simulink model "TractorTransmissionTradeOff"  (R2025a)
settings: Solver=daessc  StartTime=0.0  StopTime=125  RelTol=1e-3  AbsTol=1e-3
PreLoadFcn:
  | distanceVector = [0,0.1389,0.4167,0.8333,1.3889,2.0833,2.9167,3.889,5,6.25,7.6389,200];
  | targetVelocityVector = [0,0.5,1,1.5,2,2.5,3,3.5,4,4.5,5,5];
InitFcn:
  | TractorEnergyComputationInput
undefined symbols (not defined in the file or in its folder): engine, implement, tc, tire, tk, tphi, tykc, tykphi, tyn
libraries: nesl_utility x33, fl_lib x18, sdl_lib x6, simulink x5, slpidlib x1
(part 3 of 3)

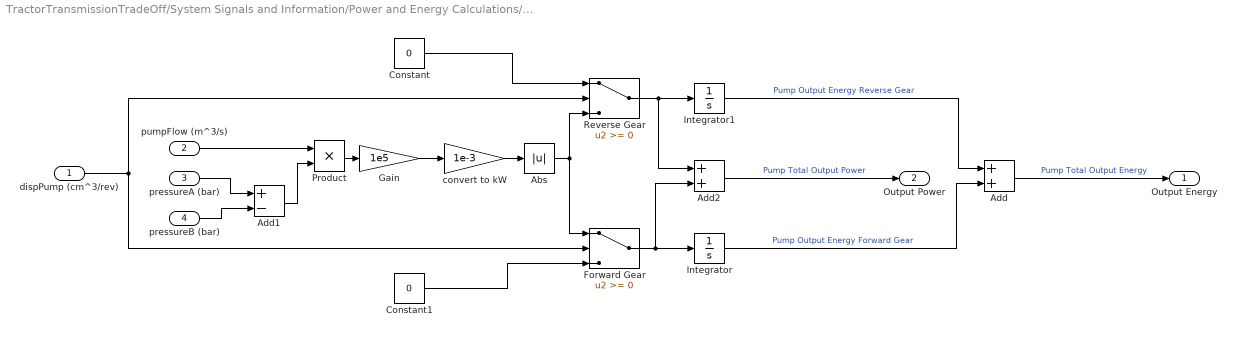
== system TractorTransmissionTradeOff/System Signals and Information/Power and Energy Calculations/Pump Computation/Pump Output Energy Computation ==
  dispPump (cm^3/rev) : Inport
  pumpFlow (m^3/s) : Inport  Port=2
  pressureA (bar) : Inport  Port=3
  pressureB (bar) : Inport  Port=4
  Abs : Abs  ZeroCross=off  SaturateOnIntegerOverflow=off
  Add : Sum
  Add1 : Sum  Inputs=+-
  Add2 : Sum
  Constant : Constant  Value=0
  Constant1 : Constant  Value=0
  Forward Gear : Switch  SaturateOnIntegerOverflow=off  InputSameDT=off
  Gain : Gain  Gain=1e5
  Integrator : Integrator
  Integrator1 : Integrator
  Product : Product
  Reverse Gear : Switch  SaturateOnIntegerOverflow=off  InputSameDT=off
  convert to kW : Gain  Gain=1e-3
  Output Energy : Outport
  Output Power : Outport  Port=2
  wires:
  pumpFlow (m^3/s)/1 -> Product/1
  Product/1 -> Gain/1
  dispPump (cm^3/rev)/1 -> Reverse Gear/2, Forward Gear/2
  Constant/1 -> Reverse Gear/1
  Constant1/1 -> Forward Gear/3
  Reverse Gear/1 -> Integrator1/1, Add2/1
  Forward Gear/1 -> Integrator/1, Add2/2
  Integrator1/1 -> Add/1  "Pump Output Energy Reverse Gear"
  Integrator/1 -> Add/2  "Pump Output Energy Forward Gear"
  Add/1 -> Output Energy/1  "Pump Total Output Energy"
  pressureA (bar)/1 -> Add1/1
  pressureB (bar)/1 -> Add1/2
  Add1/1 -> Product/2
  Gain/1 -> convert to kW/1
  Abs/1 -> Forward Gear/1, Reverse Gear/3
  convert to kW/1 -> Abs/1
  Add2/1 -> Output Power/1  "Pump Total Output Power"

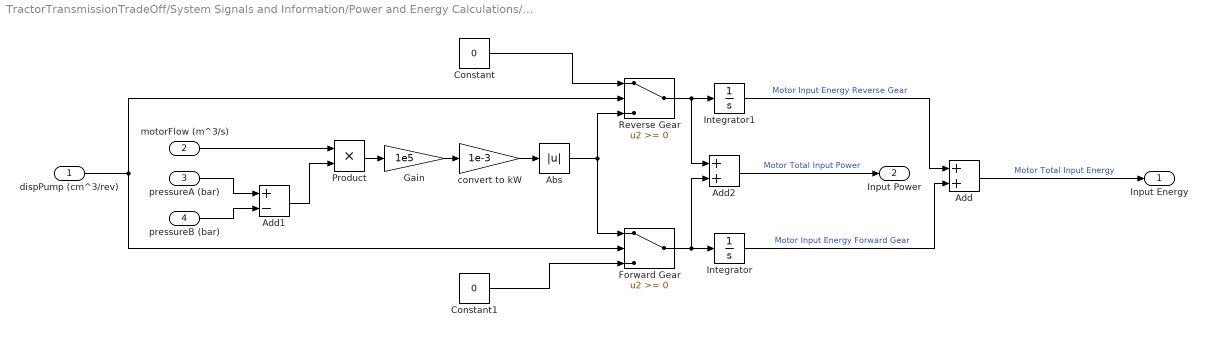
== system TractorTransmissionTradeOff/System Signals and Information/Power and Energy Calculations/Rear Motor Computation/Motor Input Energy Computation ==
  dispPump (cm^3/rev) : Inport
  motorFlow (m^3/s) : Inport  Port=2
  pressureA (bar) : Inport  Port=3
  pressureB (bar) : Inport  Port=4
  Abs : Abs  SaturateOnIntegerOverflow=off
  Add : Sum
  Add1 : Sum  Inputs=+-
  Add2 : Sum
  Constant : Constant  Value=0
  Constant1 : Constant  Value=0
  Forward Gear : Switch  SaturateOnIntegerOverflow=off  InputSameDT=off
  Gain : Gain  Gain=1e5
  Integrator : Integrator
  Integrator1 : Integrator
  Product : Product
  Reverse Gear : Switch  SaturateOnIntegerOverflow=off  InputSameDT=off
  convert to kW : Gain  Gain=1e-3
  "Input Energy " : Outport
  Input Power : Outport  Port=2
  wires:
  motorFlow (m^3/s)/1 -> Product/1
  Product/1 -> Gain/1
  dispPump (cm^3/rev)/1 -> Forward Gear/2, Reverse Gear/2
  Constant/1 -> Reverse Gear/1
  Constant1/1 -> Forward Gear/3
  Reverse Gear/1 -> Add2/1, Integrator1/1
  Forward Gear/1 -> Add2/2, Integrator/1
  Integrator1/1 -> Add/1  "Motor Input Energy Reverse Gear"
  Integrator/1 -> Add/2  "Motor Input Energy Forward Gear"
  Add/1 -> "Input Energy "/1  "Motor Total Input Energy"
  pressureA (bar)/1 -> Add1/1
  pressureB (bar)/1 -> Add1/2
  Add1/1 -> Product/2
  Abs/1 -> Forward Gear/1, Reverse Gear/3
  Gain/1 -> convert to kW/1
  convert to kW/1 -> Abs/1
  Add2/1 -> Input Power/1  "Motor Total Input Power"

== system TractorTransmissionTradeOff/System Signals and Information/Power and Energy Calculations/Rear Motor Computation/Motor Output Energy Computation ==
  wTransmission (rpm) : Inport
  tTransmission (N*m) : Inport  Port=2
  dispPump (cm^3/rev) : Inport  Port=3
  Abs : Abs  ZeroCross=off  SaturateOnIntegerOverflow=off
  Add : Sum
  Add1 : Sum
  Constant : Constant  Value=0
  Constant1 : Constant  Value=0
  Forward Gear : Switch  SaturateOnIntegerOverflow=off  InputSameDT=off
  Gain : Gain  Gain=2*pi/60
  Integrator : Integrator
  Integrator1 : Integrator
  Product : Product
  Reverse Gear : Switch  SaturateOnIntegerOverflow=off  InputSameDT=off
  convert to kW : Gain  Gain=1e-3
  Output Energy : Outport
  Output Power : Outport  Port=2
  wires:
  Gain/1 -> Product/1
  tTransmission (N*m)/1 -> Product/2
  wTransmission (rpm)/1 -> Gain/1
  dispPump (cm^3/rev)/1 -> Reverse Gear/2, Forward Gear/2
  Constant/1 -> Reverse Gear/1
  Constant1/1 -> Forward Gear/3
  Reverse Gear/1 -> Add1/1, Integrator1/1
  Forward Gear/1 -> Add1/2, Integrator/1
  Integrator1/1 -> Add/1  "Motor Output Energy Reverse Gear"
  Integrator/1 -> Add/2  "Motor Output Energy Forward Gear"
  Add/1 -> Output Energy/1  "Motor Total Output Energy"
  Product/1 -> convert to kW/1
  Abs/1 -> Forward Gear/1, Reverse Gear/3
  convert to kW/1 -> Abs/1
  Add1/1 -> Output Power/1  "Motor Total Output Power"

== system TractorTransmissionTradeOff/Tractor/Tractor Body and Powertrain/Speed Source - Engine/Sensor Engine ==
  MRRef : fl_lib/Mechanical/Rotational Elements/Mechanical Rotational Reference
  Motion Sensor : fl_lib/Mechanical/Mechanical Sensors/Ideal Rotational Motion Sensor  reference=foundation.enum.MeasurementReference.difference  acceleration_port=false  velocity_port=true  position_port=true  wrap_angle=simscape.enum.onoff.off  offset=0 rad
  PS Terminator : fl_lib/Physical Signals/Sinks/PS Terminator
  PS-Simulink Converter : nesl_utility/PS-Simulink Converter  PhysicalDomain=network_engine_domain  SubClassName=ps_output  LeftPortType=input  RightPortType=output  PseudoPeriodic=off  Frequencies=[]  VectorFormat=1-D array  Unit=rpm  AffineConversion=off
  PS2S : nesl_utility/PS-Simulink Converter  PhysicalDomain=network_engine_domain  SubClassName=ps_output  LeftPortType=input  RightPortType=output  PseudoPeriodic=off  Frequencies=[]  VectorFormat=1-D array  Unit=N*m  AffineConversion=off
  Torque Sensor : fl_lib/Mechanical/Mechanical Sensors/Ideal Torque Sensor
  A : PMIOPort  Side=Left
  B : PMIOPort  Port=2  Side=Right
  Bus Element Out : Outport  PortName=engine  Element=engineSpeed
  Bus Element Out1 : Outport  PortName=engine  Element=engineTorque
  wires:
  PS2S/1 -> Bus Element Out1/1
  PS-Simulink Converter/1 -> Bus Element Out/1
  connections:
  Torque Sensor/LConn1 -- A/RConn1 -- Motion Sensor/LConn1
  Motion Sensor/RConn2 -- PS-Simulink Converter/LConn1
  MRRef/LConn1 -- Motion Sensor/RConn1
  Torque Sensor/RConn2 -- PS2S/LConn1
  B/RConn1 -- Torque Sensor/RConn1
  Motion Sensor/RConn3 -- PS Terminator/LConn1
